simulink model "Lab2_VM_Uneven_Wall"  (R2026a)
settings: Solver=FixedStepAuto  StopTime=inf
model workspace (MAT data in the model file):
  SL_ROS_VariableLengthArrays_MaxSizes.CommonInfo.ArrayTruncateAction = 'EmitWarning'
  SL_ROS_VariableLengthArrays_MaxSizes.MsgTypeMap = containers.Map
  SL_ROS_VariableLengthArrays_MaxSizes.MsgTypeMap.serialization.keys = {'sensor_msgs/LaserScan'}
  SL_ROS_VariableLengthArrays_MaxSizes.MsgTypeMap.serialization.values{1}(1).PropertyName = 'Intensities'
  SL_ROS_VariableLengthArrays_MaxSizes.MsgTypeMap.serialization.values{1}(1).DataType = 'single'
  SL_ROS_VariableLengthArrays_MaxSizes.MsgTypeMap.serialization.values{1}(1).MaxLength = 360
  SL_ROS_VariableLengthArrays_MaxSizes.MsgTypeMap.serialization.values{1}(2).PropertyName = 'Ranges'
  SL_ROS_VariableLengthArrays_MaxSizes.MsgTypeMap.serialization.values{1}(2).DataType = 'single'
  SL_ROS_VariableLengthArrays_MaxSizes.MsgTypeMap.serialization.values{1}(2).MaxLength = 360
  SL_ROS_VariableLengthArrays_MaxSizes.MsgTypeMap.serialization.uniformity = 0
  SL_ROS_VariableLengthArrays_MaxSizes.MsgTypeMap.serialization.keyType = 'char'
  SL_ROS_VariableLengthArrays_MaxSizes.MsgTypeMap.serialization.valueType = 'any'
undefined symbols (not defined in the file or in its folder): Angular, Linear
libraries: robotlib x4
settings Model: Creator=Sina  LastModifiedBy=juulg
settings HardwareCC: ProdHWDeviceType=Generic->Unspecified (assume 32-bit Generic)  UseEmbeddedCoderFeatures=off
settings RTWCC: SystemTargetFile=ert.tlc  HardwareBoard=Robot Operating System (ROS)  TLCOptions="-aInlineSetEventsForThisBaseRateFcn=TLC_FALSE -aSuppressMultiTaskScheduler=TLC_FALSE  -aRateBasedStepFcn=0"  Toolchain=Catkin  TargetLang=C++  Description=Embedded Coder
settings ERTTargetCC: SupportNonInlinedSFcns=on

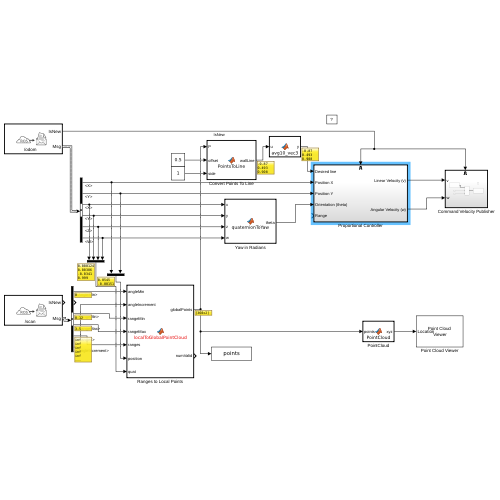
[thumbnail: Simulink's stored preview of the top-level diagram]
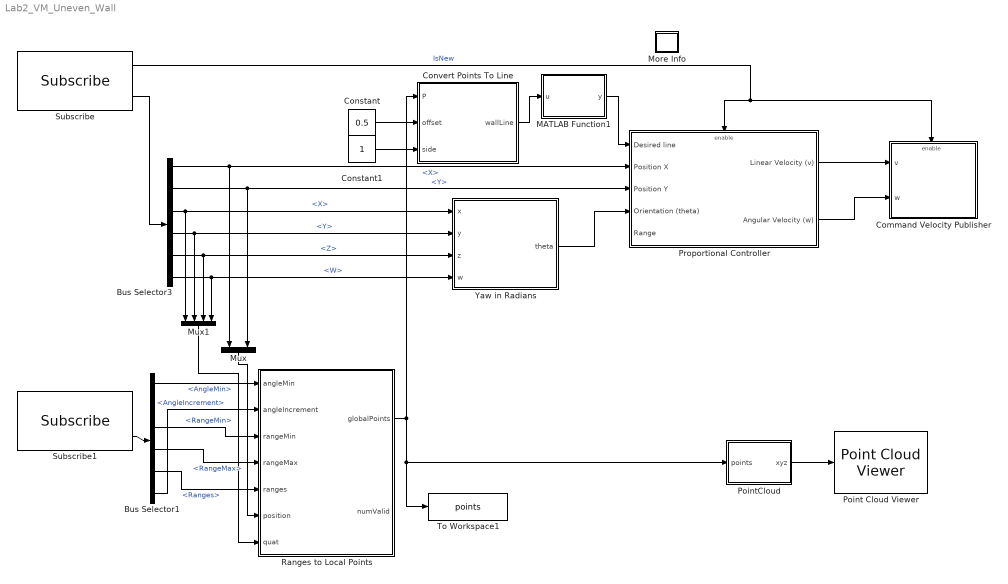
== system Lab2_VM_Uneven_Wall ==
  Bus Selector1 : BusSelector  OutputSignals=AngleMin,AngleMax,RangeMin,RangeMax,Ranges,AngleIncrement
  Bus Selector3 : BusSelector  OutputSignals=Pose.Pose.Position.X,Pose.Pose.Position.Y,Pose.Pose.Orientation.X,Pose.Pose.Orientation.Y,Pose.Pose.Orientation.Z,Pose.Pose.Orientation.W
  Command Velocity Publisher : Subsystem
  Constant : Constant  Value=0.5
  Constant1 : Constant
  Convert Points To Line : MATLAB Function  TreatAsAtomicUnit=on
  MATLAB Function1 : MATLAB Function  TreatAsAtomicUnit=on
  More Info : Subsystem
      settings: OpenFcn=showdemo(bdroot(gcb))
      mask Display: disp('?')
  Mux : Mux  Inputs=2
  Mux1 : Mux
  Point Cloud Viewer : PointCloudViewer  FigPos=[3843 1177 1916 1112]  FigSettingsValue=[-7.58662079218697 28.9349744574912 -10.400794325611 5.29998510606108 -1 1 1]
  PointCloud : MATLAB Function  TreatAsAtomicUnit=on
  Proportional Controller : Subsystem
  Ranges to Local Points : MATLAB Function  TreatAsAtomicUnit=on
  Subscribe : robotlib/Subscribe  topicSource=Select from ROS network  topic=/odom  messageType=nav_msgs/Odometry  SampleTime=-1  legacyBusStruct=off  messageQueueLength=51
  Subscribe1 : robotlib/Subscribe  topicSource=Select from ROS network  topic=/scan  messageType=sensor_msgs/LaserScan  SampleTime=-1  legacyBusStruct=off  messageQueueLength=51
  To Workspace1 : ToWorkspace  VariableName=points  SaveFormat=Timeseries  SampleTime=-1
  Yaw in Radians : MATLAB Function  TreatAsAtomicUnit=on
  wires:
  Proportional Controller/2(Angular Velocity (w)) -> Command Velocity Publisher/2(w)
  Subscribe/1 -> Command Velocity Publisher/Enable, Proportional Controller/Enable  "IsNew"
  Proportional Controller/1(Linear Velocity (v)) -> Command Velocity Publisher/1(v)
  Subscribe/2 -> Bus Selector3/1
  Subscribe1/2 -> Bus Selector1/1
  Bus Selector3/3 -> Yaw in Radians/1(x), Mux1/1  "<X>"
  Bus Selector3/4 -> Yaw in Radians/2(y), Mux1/2  "<Y>"
  Bus Selector3/5 -> Yaw in Radians/3(z), Mux1/3  "<Z>"
  Bus Selector3/6 -> Yaw in Radians/4(w), Mux1/4  "<W>"
  Bus Selector3/1 -> Proportional Controller/2(Position X), Mux/1  "<X>"
  Bus Selector3/2 -> Proportional Controller/3(Position Y), Mux/2  "<Y>"
  Yaw in Radians/1(theta) -> Proportional Controller/4(Orientation (theta))
  PointCloud/1(xyz) -> Point Cloud Viewer/1
  Convert Points To Line/1(wallLine) -> MATLAB Function1/1(u)
  MATLAB Function1/1(y) -> Proportional Controller/1(Desired line)
  Constant/1 -> Convert Points To Line/2(offset)
  Constant1/1 -> Convert Points To Line/3(side)
  Bus Selector1/1 -> Ranges to Local Points/1(angleMin)  "<AngleMin>"
  Bus Selector1/3 -> Ranges to Local Points/3(rangeMin)  "<RangeMin>"
  Bus Selector1/4 -> Ranges to Local Points/4(rangeMax)  "<RangeMax>"
  Bus Selector1/5 -> Ranges to Local Points/5(ranges)  "<Ranges>"
  Mux/1 -> Ranges to Local Points/6(position)
  Mux1/1 -> Ranges to Local Points/7(quat)
  Ranges to Local Points/1(globalPoints) -> PointCloud/1(points), To Workspace1/1, Convert Points To Line/1(P)
  Bus Selector1/6 -> Ranges to Local Points/2(angleIncrement)  "<AngleIncrement>"

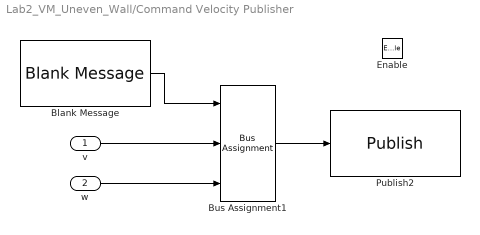
== system Lab2_VM_Uneven_Wall/Command Velocity Publisher ==
  v : Inport
  w : Inport  Port=2
  Enable : EnablePort
  Blank Message : robotlib/Blank Message  messageClass=Message  entityType=geometry_msgs/Twist  messageType=geometry_msgs/Twist  SampleTime=inf  legacyBusStruct=off
  Bus Assignment1 : BusAssignment  DialogController=Simulink.DDGSource_BusAssignment  AssignedSignals=Linear.X,Angular.Z
  Publish2 : robotlib/Publish  topicSource=Select from ROS network  topic=/cmd_vel  messageType=geometry_msgs/Twist  legacyBusStruct=off  messageQueueLength=105
  wires:
  Bus Assignment1/1 -> Publish2/1
  Blank Message/1 -> Bus Assignment1/1
  v/1 -> Bus Assignment1/2
  w/1 -> Bus Assignment1/3

== system Lab2_VM_Uneven_Wall/More Info ==

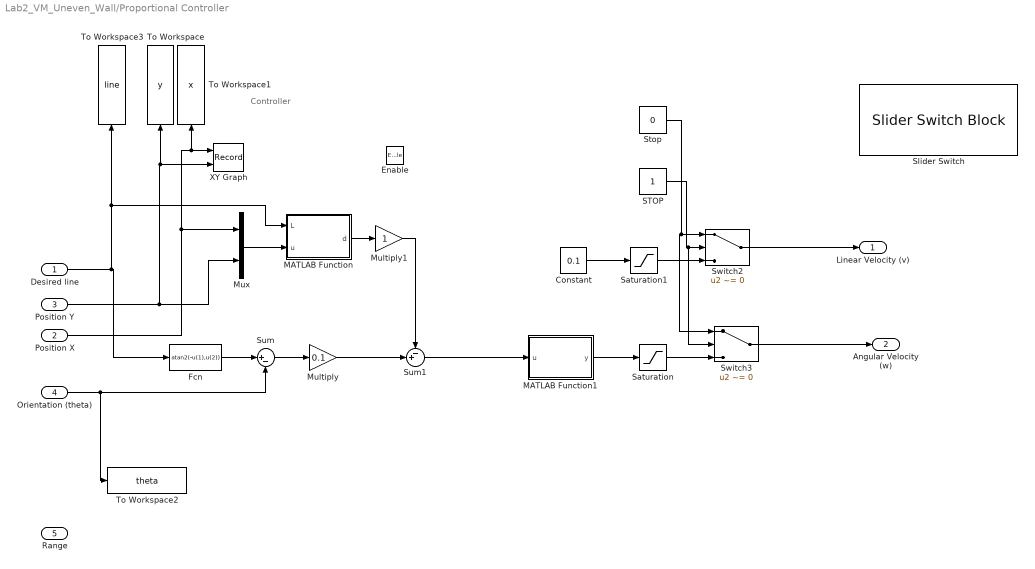
== system Lab2_VM_Uneven_Wall/Proportional Controller ==
  note: Controller
  Desired line : Inport
  Position X : Inport  Port=2
  Position Y : Inport  Port=3
  Orientation (theta) : Inport  Port=4
  Range : Inport  Port=5
  Enable : EnablePort
  Constant : Constant  Value=0.1
  Fcn : Fcn  Expr=atan2(-u(1),u(2))
  MATLAB Function : MATLAB Function  TreatAsAtomicUnit=on
  MATLAB Function1 : MATLAB Function  TreatAsAtomicUnit=on
  Multiply : Gain  Gain=0.1
  Multiply1 : Gain
  Mux : Mux  Inputs=2
  "STOP " : Constant
  Saturation : Saturate  UpperLimit=2.84  LowerLimit=-2.84
  Saturation1 : Saturate  UpperLimit=0.22  LowerLimit=-0.22
  Slider Switch : SliderSwitchBlock
  Stop : Constant  Value=0
  Sum : Sum  Inputs=|+-
  Sum1 : Sum  Inputs=-+|
  Switch2 : Switch  Criteria=u2 ~= 0  SaturateOnIntegerOverflow=off  InputSameDT=off
  Switch3 : Switch  Criteria=u2 ~= 0  SaturateOnIntegerOverflow=off  InputSameDT=off
  To Workspace : ToWorkspace  VariableName=y  SaveFormat=Timeseries  SampleTime=-1
  To Workspace1 : ToWorkspace  VariableName=x  SaveFormat=Timeseries  SampleTime=-1
  To Workspace2 : ToWorkspace  VariableName=theta  SaveFormat=Timeseries  SampleTime=-1
  To Workspace3 : ToWorkspace  VariableName=line  SaveFormat=Timeseries  SampleTime=-1
  XY Graph : Record  NumPorts=2.0  FileSettingsInternal="{\"entries\":[{\"content\":{\"excelSettings\":{\"content\":{},\"type\":\"Streamout.ExcelSettings\"},\"parquetSettings\":{\"content\":{},\"type\":\"Streamout.ParquetSettings\"}},\"type\":\"Streamout.FileSettingStorage\",\"uuid\":\"\"}],\"packageUris\":[\"http:\\/\\/schema.mathworks.com\\/mf0\\/streamout_blocks\\/R2020a\"],\"version\":\"1.0\"}"  FrameSettings=[0, 0]  Layout=[1 1]  SignalsInternal="{\"entries\":[{\"content\":{\"signals\":[{\"content\":{\"blockPath\":[],\"dimensions\":[1],\"domain\":\"\",\"lineColor\":\"#a2142f\",\"plots\":[ 1 ],\"port\":1,\"sid\":[\"\"],\"signalID\":1,\"signalName\":\"X\"},\"type\":\"RecordBlkView.Signal\",\"uuid\":\"\"},{\"content\":{\"blockPath\":[],\"dimensions\":[1],\"domain\":\"\",\"lineColor\":\"#139fff\",\"plots\":[ 1 ],\"port\":2,\"sid\":[\"\"],\"signalID\":2,\"signalName\":\"Y\"},\"type\":\"RecordBlkView.Signal\",\"uuid\":\"\"}]},\"type\":\"RecordBlkView.InputSignals\",\"uuid\":\"\"}],\"packageUris\":[\"http:\\/\\/schema.mathworks.com\\/mf0\\/streamout_blocks\\/R2020a\"],\"version\":\"1.0\"}"  VisualizationBindings="{\"xyplotplugin\":{\"info\":[{\"series\":[{\"bindingParametersList\":[{\"parameter\":\"X-Axis\",\"signalID\":1,\"signalName\":\"X\"},{\"parameter\":\"Y-Axis\",\"signalID\":2,\"signalName\":\"Y\"}],\"seriesID\":0}],\"subplotID\":1}]}}"  CompatibilityTag=XY
  Linear Velocity (v) : Outport  VectorParamsAs1DForOutWhenUnconnected=off
  Angular Velocity (w) : Outport  Port=2  VectorParamsAs1DForOutWhenUnconnected=off
  wires:
  Stop/1 -> Switch3/1, Switch2/1
  "STOP "/1 -> Switch3/2, Switch2/2
  Switch2/1 -> Linear Velocity (v)/1
  Switch3/1 -> Angular Velocity (w)/1
  Mux/1 -> MATLAB Function/2(u)
  Multiply1/1 -> Sum1/1
  Position Y/1 -> To Workspace/1, XY Graph/2, Mux/2
  Position X/1 -> Mux/1, To Workspace1/1, XY Graph/1
  Desired line/1 -> Fcn/1, MATLAB Function/1(L), To Workspace3/1
  Sum/1 -> Multiply/1
  Multiply/1 -> Sum1/2
  Fcn/1 -> Sum/1
  MATLAB Function/1(d) -> Multiply1/1
  Orientation (theta)/1 -> To Workspace2/1, Sum/2
  Constant/1 -> Saturation1/1
  Sum1/1 -> MATLAB Function1/1(u)
  Saturation/1 -> Switch3/3
  Saturation1/1 -> Switch2/3
  MATLAB Function1/1(y) -> Saturation/1

== matlab function Lab2_VM_Uneven_Wall/PointCloud ==
  data: points input; xyz output
function xyz = PointCloud(points)
xyz = [points, zeros(size(points, 1), 1)];
end

== matlab function Lab2_VM_Uneven_Wall/Proportional Controller/MATLAB Function1 ==
  data: u input; y output
function y = fcn(u)
    if isnan(u)
        u=0;
    end
    y = u;
end

== matlab function Lab2_VM_Uneven_Wall/Yaw in Radians ==
  data: x input; theta output; y input; z input; w input
function theta = quaternionToYaw(x,y,z,w)

    theta = atan2(2*(w*z + x*y), ...
                  1 - 2*(y*y + z*z));

end

== matlab function Lab2_VM_Uneven_Wall/Ranges to Local Points ==
  data: angleMin input; angleIncrement input; rangeMin input; rangeMax input; ranges input; globalPoints output; position input; quat input; numValid output
function [globalPoints, numValid] = localToGlobalPointCloud(angleMin, angleIncrement, rangeMin, rangeMax, ranges, position, quat)
    % Returns a fixed-size N-by-2 matrix (N = numel(ranges)).
    % Invalid beams (NaN, Inf, out of range) are set to NaN instead of removed.
    
    robotX = position(1);
    robotY = position(2);
    quatX = quat(1);
    quatY = quat(2);
    quatZ = quat(3);
    quatW = quat(4);
    
    r = double(ranges(:));
    n = numel(r);
    
    yaw = atan2(2*(quatW*quatZ + quatX*quatY), ...
    1 - 2*(quatY^2 + quatZ^2));
    
    angles = angleMin + (0:n-1)' * angleIncrement;
    
    valid = isfinite(r) & (r >= rangeMin) & (r <= rangeMax);
    r(~valid) = NaN;
    
    localX = r .* cos(angles);
    localY = r .* sin(angles);
    
    globalX = robotX + cos(yaw)*localX - sin(yaw)*localY;
    globalY = robotY + sin(yaw)*localX + cos(yaw)*localY;
    
    globalPoints = [globalX, globalY];   % n-by-2, fixed size
    numValid = sum(valid);
end

== matlab function Lab2_VM_Uneven_Wall/Convert Points To Line ==
  data: P input; wallLine output; offset input; side input
function wallLine = PointsToLine(P, offset, side)
% P      : Nx2 points (any numeric type)
% offset : desired wall distance [m]
% side   : -1 = wall on the right, +1 = wall on the left
% wallLine : [a b c], real double, a*x + b*y + c = 0, sqrt(a^2+b^2) = 1

    P      = double(P);
    offset = double(offset);
    side   = double(side);

    wallLine = zeros(1, 3);

    valid = all(isfinite(P), 2);
    cnt = sum(valid);
    if cnt < 2
        return;                      % no wall found: [0 0 0]
    end

    Pv = P;
    Pv(~valid, :) = 0;
    m = sum(Pv, 1) / cnt;            % mean of valid points

    D = P - m;
    D(~valid, :) = 0;

    % Covariance terms
    Sxx = sum(D(:,1).^2) / cnt;
    Syy = sum(D(:,2).^2) / cnt;
    Sxy = sum(D(:,1).*D(:,2)) / cnt;

    % Principal direction of a 2x2 covariance (closed form, always real)
    theta = 0.5 * atan2(2*Sxy, Sxx - Syy);
    d = [cos(theta), sin(theta)];    % unit wall direction

    % Orient along the robot's forward axis (+x)
    if d(1) < 0 || (abs(d(1)) < 1e-9 && d(2) < 0)
        d = -d;
    end

    nL = [-d(2), d(1)];              % unit normal pointing left
    m2 = m - side * offset * nL;     % point on the offset line

    wallLine(1) = nL(1);
    wallLine(2) = nL(2);
    wallLine(3) = -(nL(1)*m2(1) + nL(2)*m2(2));
end

== matlab function Lab2_VM_Uneven_Wall/Proportional Controller/MATLAB Function ==
  data: L input; u input; d output
function d = LineDist(L,u)
d= (u(1)*L(1)+u(2)*L(2)+L(3))/sqrt(L(1)^2+L(2)^2);

== matlab function Lab2_VM_Uneven_Wall/MATLAB Function1 ==
  data: u input; y output
function y = avg10_vec3(u)
len = 50;
% u must be a 3x1 column vector
persistent buf idx count
if isempty(buf)
    buf = zeros(3, len);
    idx = 1;
    count = 0;
end
buf(:, idx) = u(:);
idx = mod(idx, len) + 1;
count = min(count + 1, len);
y = sum(buf(:, 1:count), 2) / count;
end
